simulink subsystem "FlexibleDriveline"  (R2025b)
settings: Solver=VariableStepAuto  StartTime=0.0  StopTime=10.0  RelTol=1e-3
PreLoadFcn:
  | FlexibleDrivelineParams;
undefined symbols (not defined in the file or in its folder): flexDLParams, fs
libraries: fl_lib x41, sdl_lib x24, nesl_utility x3
(part 2 of 2)

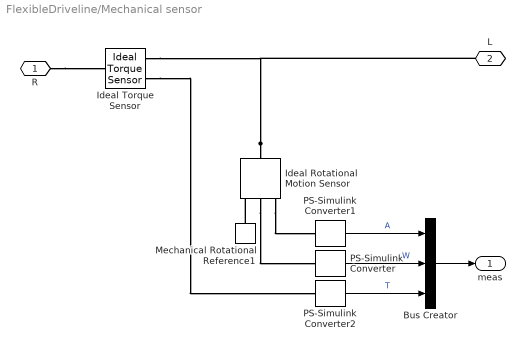
== system FlexibleDriveline/Mechanical sensor ==
  Bus Creator : BusCreator  Inputs=3
  Ideal Rotational Motion Sensor : fl_lib/Mechanical/Mechanical Sensors/Ideal Rotational Motion Sensor  reference=foundation.enum.MeasurementReference.difference  acceleration_port=false  velocity_port=true  position_port=true  wrap_angle=simscape.enum.onoff.off  offset=0 deg
  Ideal Torque Sensor : fl_lib/Mechanical/Mechanical Sensors/Ideal Torque Sensor
  Mechanical Rotational Reference1 : fl_lib/Mechanical/Rotational Elements/Mechanical Rotational Reference
  PS-Simulink Converter : nesl_utility/PS-Simulink Converter  PhysicalDomain=network_engine_domain  SubClassName=ps_output  LeftPortType=input  RightPortType=output  PseudoPeriodic=off  Frequencies=[]  VectorFormat=1-D array  Unit=rad/s  AffineConversion=off
  PS-Simulink Converter1 : nesl_utility/PS-Simulink Converter  PhysicalDomain=network_engine_domain  SubClassName=ps_output  LeftPortType=input  RightPortType=output  PseudoPeriodic=off  Frequencies=[]  VectorFormat=1-D array  Unit=rad  AffineConversion=off
  PS-Simulink Converter2 : nesl_utility/PS-Simulink Converter  PhysicalDomain=network_engine_domain  SubClassName=ps_output  LeftPortType=input  RightPortType=output  PseudoPeriodic=off  Frequencies=[]  VectorFormat=1-D array  Unit=N*m  AffineConversion=off
  R : PMIOPort  Side=Left
  L : PMIOPort  Port=2  Side=Right
  meas : Outport  VectorParamsAs1DForOutWhenUnconnected=off
  wires:
  PS-Simulink Converter2/1 -> Bus Creator/3  "T"
  PS-Simulink Converter/1 -> Bus Creator/2  "W"
  PS-Simulink Converter1/1 -> Bus Creator/1  "A"
  Bus Creator/1 -> meas/1
  connections:
  Mechanical Rotational Reference1/LConn1 -- Ideal Rotational Motion Sensor/RConn1
  Ideal Rotational Motion Sensor/RConn3 -- PS-Simulink Converter1/LConn1
  Ideal Rotational Motion Sensor/RConn2 -- PS-Simulink Converter/LConn1
  Ideal Rotational Motion Sensor/LConn1 -- Ideal Torque Sensor/RConn1 -- L/RConn1
  R/RConn1 -- Ideal Torque Sensor/LConn1
  Ideal Torque Sensor/RConn2 -- PS-Simulink Converter2/LConn1

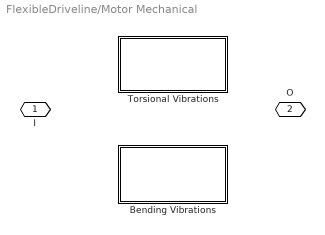
== system FlexibleDriveline/Motor Mechanical ==
  Bending Vibrations : Subsystem  VariantControl=false
  Torsional Vibrations : Subsystem  VariantControl=true
  I : PMIOPort  Side=Left
  O : PMIOPort  Port=2  Side=Right

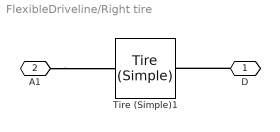
== system FlexibleDriveline/Right tire ==
  Tire (Simple)1 : sdl_lib/Tires & Vehicles/Tire (Simple)  r_tire=flexDLParams.gearBox.tireR m  model_compliance=sdl.enum.compliance.on  stiffness=1e6 N/m  damping=1000 N*s/m  model_inertia=sdl.enum.model_inertia.on  tire_inertia=1 kg*m^2  initial_velocity=0 rad/s
      settings: InternalSimscapePortConfiguration="{\"Bottom\":[],\"Left\":[{\"id\":\"A\",\"label\":\"A\",\"type\":\"foundation.mechanical.rotational.rotational\"}],\"Right\":[{\"id\":\"H\",\"label\":\"H\",\"type\":\"foundation.mechanical.translational.translational\"}],\"Top\":[]}"
  D : PMIOPort  Side=Left
  A1 : PMIOPort  Port=2  Side=Right
  connections:
  A1/RConn1 -- Tire (Simple)1/LConn1
  D/RConn1 -- Tire (Simple)1/RConn1

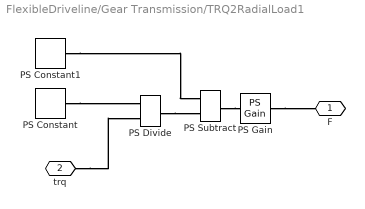
== system FlexibleDriveline/Gear Transmission/TRQ2RadialLoad1 ==
  PS Constant : fl_lib/Physical Signals/Sources/PS Constant  constant=25e-3 m
  PS Constant1 : fl_lib/Physical Signals/Sources/PS Constant  constant=5*9.81 N
  PS Divide : fl_lib/Physical Signals/Functions/PS Divide
  PS Gain : fl_lib/Physical Signals/Functions/PS Gain  gain=0.5
  PS Subtract : fl_lib/Physical Signals/Functions/PS Subtract
  F : PMIOPort  Side=Right
  trq : PMIOPort  Port=2  Side=Left
  connections:
  trq/RConn1 -- PS Divide/LConn1
  PS Constant1/RConn1 -- PS Subtract/LConn2
  PS Divide/RConn1 -- PS Subtract/LConn1
  PS Gain/RConn1 -- F/RConn1
  PS Subtract/RConn1 -- PS Gain/LConn1
  PS Constant/RConn1 -- PS Divide/LConn2

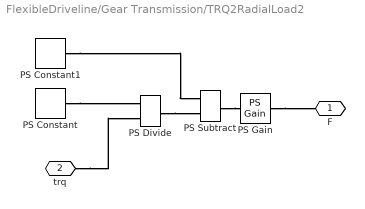
== system FlexibleDriveline/Gear Transmission/TRQ2RadialLoad2 ==
  PS Constant : fl_lib/Physical Signals/Sources/PS Constant  constant=25e-3 m
  PS Constant1 : fl_lib/Physical Signals/Sources/PS Constant  constant=5*9.81 N
  PS Divide : fl_lib/Physical Signals/Functions/PS Divide
  PS Gain : fl_lib/Physical Signals/Functions/PS Gain  gain=0.5
  PS Subtract : fl_lib/Physical Signals/Functions/PS Subtract
  F : PMIOPort  Side=Right
  trq : PMIOPort  Port=2  Side=Left
  connections:
  trq/RConn1 -- PS Divide/LConn1
  PS Constant1/RConn1 -- PS Subtract/LConn2
  PS Divide/RConn1 -- PS Subtract/LConn1
  PS Gain/RConn1 -- F/RConn1
  PS Subtract/RConn1 -- PS Gain/LConn1
  PS Constant/RConn1 -- PS Divide/LConn2

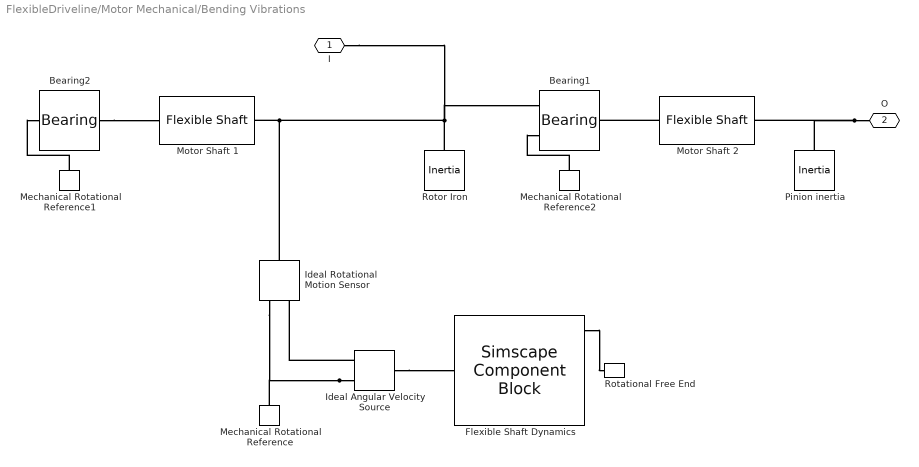
== system FlexibleDriveline/Motor Mechanical/Bending Vibrations ==
  Bearing1 : sdl_lib/Couplings & Drives/Bearing  bearingType=sdl.enum.bearingType.BallRoller  enableFollower=true  casing=true  radius=flexDLParams.motorMech.bearing1ID/2 mm  length=flexDLParams.motorMech.bearing1Length mm  loadType=foundation.enum.constant_variable.constant  load=10 N  F_thr=0.001 N  w_thr=0.001 rev/s  frictionType=foundation.enum.constant_variable.variable  interp_method_1=simscape.enum.interpolation.linear  extrap_method_1=simscape.enum.extrapolation.linear  f_coeff=0.002  N_TLU=flexDLParams.motorMech.speedRPM rpm  f_coeff_TLU=flexDLParams.motorMech.frictionCoff  customizeFrictionCurve=false  mu=0.29 Pa*s  visc_coeff_min=0.002  bearingModulus=7.2519e-08 rev  muN_P_norm_TLU=[.4306, .6124, .6651, .7512, .866, 1, 1.1962, 1.4354, 3.8517]  visc_coeff_norm_TLU=[3.6621, 1.672, 1.3397, 1.1811, 1.0743, 1, 1.0358, 1.1173, 2.2792]  interp_method_2=simscape.enum.interpolation.linear  extrap_method_2=simscape.enum.extrapolation.linear
      settings: InternalSimscapePortConfiguration="{\"Bottom\":[{\"id\":\"C\",\"label\":\"C\",\"type\":\"foundation.mechanical.rotational.rotational\"}],\"Left\":[{\"id\":\"B\",\"label\":\"B\",\"type\":\"foundation.mechanical.rotational.rotational\"}],\"Right\":[{\"id\":\"F\",\"label\":\"F\",\"type\":\"foundation.mechanical.rotational.rotational\"}],\"Top\":[]}"
  Bearing2 : sdl_lib/Couplings & Drives/Bearing  bearingType=sdl.enum.bearingType.BallRoller  enableFollower=false  casing=true  radius=flexDLParams.motorMech.bearing2ID/2 mm  length=flexDLParams.motorMech.bearing1Length mm  loadType=foundation.enum.constant_variable.constant  load=10 N  F_thr=0.001 N  w_thr=0.001 rev/s  frictionType=foundation.enum.constant_variable.variable  interp_method_1=simscape.enum.interpolation.linear  extrap_method_1=simscape.enum.extrapolation.linear  f_coeff=0.002  N_TLU=flexDLParams.motorMech.speedRPM rpm  f_coeff_TLU=flexDLParams.motorMech.frictionCoff  customizeFrictionCurve=false  mu=0.29 Pa*s  visc_coeff_min=0.002  bearingModulus=7.2519e-08 rev  muN_P_norm_TLU=[.4306, .6124, .6651, .7512, .866, 1, 1.1962, 1.4354, 3.8517]  visc_coeff_norm_TLU=[3.6621, 1.672, 1.3397, 1.1811, 1.0743, 1, 1.0358, 1.1173, 2.2792]  interp_method_2=simscape.enum.interpolation.linear  extrap_method_2=simscape.enum.extrapolation.linear
      settings: InternalSimscapePortConfiguration="{\"Bottom\":[{\"id\":\"C\",\"label\":\"C\",\"type\":\"foundation.mechanical.rotational.rotational\"}],\"Left\":[{\"id\":\"B\",\"label\":\"B\",\"type\":\"foundation.mechanical.rotational.rotational\"}],\"Right\":[],\"Top\":[]}"
  Flexible Shaft Dynamics : SimscapeComponentBlock  SourceFile=sdl.couplings.flexible_shaft  ComponentPath=sdl.couplings.flexible_shaft  ComponentVariants="[\"sdl.couplings.flexible_shaft\"]"  ComponentVariantNames="[\"flexible_shaft\"]"  ClassName=flexible_shaft  SchemaVersion=1  modelTorsion=false  modelTransverse=true  n_segments=1  parameterization=sdl.enum.shaftParameterization.MaterialPropertiesVaried  length=fs.length_shaft m  lengths=fs.zShaft m  shaft_stiffness=2e5 N*m/rad  shaft_inertia=0.02 kg*m^2  shaft_stiffnesses=[400000, 200000, 100000] N*m/rad  shaft_inertias=[.025, .02, .015] kg*m^2  eiIN=5e5 Pa*m^4  rhoaIN=19 kg/m  eiINs=[600000, 500000, 400000] Pa*m^4  rhoaINs=[20, 19, 18] kg/m  density=fs.materialDensity kg/m^3  shear_modulus=fs.shear_modulus Pa  elastic_modulus=fs.elasticModulus Pa  shaft_construction=sdl.enum.shaftConstruction.solid  diameter_outer=fs.diameters_outer(1) m  diameter_inner=fs.diameters_inner(1) m  diameter_outers=fs.diametersOuterTLU m  diameter_inners=interp1(fs.z_TLU, fs.diameters_inner_TLU, fs.z_shaft(2:end)) m  damping_ratio=0.01  mu_visc_BF=[0, 0] N*m/(rad/s)  mu_visc=fs.muViscTors N*m/(rad/s)  initial_deflection=0 rad  initial_velocity=0 rpm  num_supports=sdl.enum.num_supports.two  z_support=fs.zSupport m  boundaryB1=sdl.enum.shaftSupport.bearingMatrix_speed  DrotB1_row=fs.bearing.dRot N*m/(rad/s)  DtransB1_row=[20000, -44000, -44000, 350000] N/(m/s)  DtransB1_w_mat=fs.bearing.D N/(m/s)  KrotB1_row=fs.bearing.kRot N*m/rad  KtransB1_row=[1000000, -200000, -300000, 5000000] N/m  KtransB1_w_mat=fs.bearing.K N/m  boundaryI1=sdl.enum.shaftSupport.bearingMatrix_speed  DrotI1_row=fs.bearing.d_rot N*m/(rad/s)  DtransI1_row=[20000, -44000, -44000, 350000] N/(m/s)  DtransI1_w_mat=fs.bearing.D N/(m/s)  KrotI1_row=fs.bearing.k_rot N*m/rad  KtransI1_row=[1000000, -200000, -300000, 5000000] N/m  KtransI1_w_mat=fs.bearing.K N/m  boundaryI2=sdl.enum.shaftSupport.bearingMatrix_speed  DrotI2_row=fs.bearing.d_rot N*m/(rad/s)  DtransI2_row=[20000, -44000, -44000, 350000] N/(m/s)  DtransI2_w_mat=fs.bearing.D N/(m/s)  KrotI2_row=fs.bearing.k_rot N*m/rad  KtransI2_row=[1000000, -200000, -300000, 5000000] N/m  KtransI2_w_mat=fs.bearing.K N/m  boundaryF1=sdl.enum.shaftSupport.free  DrotF1_row=fs.bearing.dRot N*m/(rad/s)  DtransF1_row=[20000, -44000, -44000, 350000] N/(m/s)  DtransF1_w_mat=fs.bearing.D N/(m/s)  KrotF1_row=fs.bearing.kRot N*m/rad  KtransF1_row=[1000000, -200000, -300000, 5000000] N/m  KtransF1_w_mat=fs.bearing.K N/m  bearing_speed=fs.bearingSpeed*fs.excitationPoles rpm  alpha=fs.aDamp 1/s  beta=fs.bDamp s  noDisk=sdl.enum.shaftDisks.disk  zDisk=fs.zMass m  mDiskIN=fs.pointMass kg  IdDiskIN=fs.Id kg*m^2  IpDiskIN=fs.Ip./fs.excitationPoles kg*m^2  enable_static_unbalance=true  offsetMR=fs.excitationLoad./(fs.excitationPoles*fs.wNominalForcing)^2 kg*m  offsetMR_initialAngleIN=0 rad  offsetMassLocation=fs.bearingSpan12/2 m  enable_external_force=false  externalForce=[1, 2] N  externalForceHarmonic=[.5, 2]  externalLoadAngle=[pi / 2, 3 * pi / 4] rad  zExternalLoad=[.25, .75] m  AnalysisMethod=sdl.enum.bendingAnalysisMethod.Eigenmodes  ModeInputMethod=sdl.enum.modeInputMethod.SimscapeDetermined  numModesIn=fs.numModes  mode_speed_dependency=sdl.enum.mode_speed_dependency.Dynamic  OmegaNom=fs.w_shaft_nominal rad/s  wMax=fs.wMax rad/s  dz=fs.dz m  userMode_w=[280, 644, 615, 1285] rad/s  userMode_w_mat=[257, 780, 580, 1560; 280, 644, 615, 1285; 294, 513, 636, 1020] rad/s  userMode_z=[0, .1, .2, .3, .4, .5, .6, .7, .8, .9, 1] m  userMode_shapeX=[.1648, .0086, -.2759, .0162; .1671, .0093, -.2231, .0133; .1691, .01, -.1689, .0102; .1707, .0105, -.1135, .007; .1717, .0108, -.057, .0035; .1721, .0109, 0, 0; .1717, .0108, .057, -.0035; .1707, .0105, .1135, -.007; .1691, .01, .1689, -.0102; .1671, .0093, .2231, -.0133; .1648, .0086, .2759, -.0162]  userMode_shapeX_mat=cat(3, [.1842, .0134, -.3072, .0272; .1863, .0152, -.2482, .0226; .1882, .0169, -.1878, .0176; .1897, .0182, -.1261, .0121; .1906, .019, -.0634, .0062; .191, .0193, 0, 0; .1906, .019, .0634, -.0062; .1897, .0182, .1261, -.0121; .1882, .0169, .1878, -.0176; .1863, .0152, .2482, -.0226; .1842, .0134, .3072, -.0272], [.1648, .0086, -.2759, .0162; .1671, .0093, -.2231, .0133; .1691, .01, -.1689, .0102; .1707, .0105, -.1135, .007; .1717, .0108, -.057, .0035; .1721, .0109, 0, 0; .1717, .0108, .057, -.0035; .1707, .0105, .1135, -.007; .1691, .01, .1689, -.0102; .1671, .0093, .2231, -.0133; .1648, .0086, .2759, -.0162], [.1291, .0046, -.2166, .0082; .131, .0048, -.1751, .0067; .1327, .005, -.1327, .0051; .1341, .0052, -.0891, .0035; .135, .0053, -.0448, .0017; .1353, .0053, 0, 0; .135, .0053, .0448, -.0017; .1341, .0052, .0891, -.0035; .1327, .005, .1327, -.0051; .131, .0048, .1751, -.0067; .1291, .0046, .2166, -.0082])  userMode_shapeY=[.1193, -.1784, -.1997, -.3348; .1209, -.1933, -.1615, -.2751; .1224, -.2068, -.1223, -.2119; .1235, -.2176, -.0821, -.1445; .1243, -.2245, -.0413, -.0734; .1246, -.2269, 0, 0; .1243, -.2245, .0413, .0734; .1235, -.2176, .0821, .1445; .1224, -.2068, .1223, .2119; .1209, -.1933, .1615, .2751; .1193, -.1784, .1997, .3348]  userMode_shapeY_mat=cat(3, [.0885, -.1625, -.1475, -.3301; .0895, -.1847, -.1192, -.2745; .0904, -.2048, -.0902, -.2141; .0911, -.2209, -.0606, -.1475; .0916, -.2313, -.0304, -.0754; .0917, -.2349, 0, 0; .0916, -.2313, .0304, .0754; .0911, -.2209, .0606, .1475; .0904, -.2048, .0902, .2141; .0895, -.1847, .1192, .2745; .0885, -.1625, .1475, .3301], [.1193, -.1784, -.1997, -.3348; .1209, -.1933, -.1615, -.2751; .1224, -.2068, -.1223, -.2119; .1235, -.2176, -.0821, -.1445; .1243, -.2245, -.0413, -.0734; .1246, -.2269, 0, 0; .1243, -.2245, .0413, .0734; .1235, -.2176, .0821, .1445; .1224, -.2068, .1223, .2119; .1209, -.1933, .1615, .2751; .1193, -.1784, .1997, .3348], [.1566, -.1901, -.2628, -.3377; .1589, -.1994, -.2125, -.2753; .161, -.2079, -.1609, -.2103; .1627, -.2146, -.1081, -.1424; .1638, -.219, -.0544, -.0719; .1642, -.2205, 0, 0; .1638, -.219, .0544, .0719; .1627, -.2146, .1081, .1424; .161, -.2079, .1609, .2103; .1589, -.1994, .2125, .2753; .1566, -.1901, .2628, .3377])  eta_lumped_nominal=5e-7  etaDer_lumped_nominal=1e-4  eta_modal_nominal=1  etaDer_modal_nominal=1
      settings: CopyFcn=simscape.sscblock.internal.componentBlockCallback(gcbh,'COPY')  PreCopyFcn=simscape.sscblock.internal.componentBlockCallback(gcbh,'PRECOPY')  PreDeleteFcn=simscape.sscblock.internal.componentBlockCallback(gcbh,'PREDELETE')  InternalSimscapePortConfiguration="{\"Bottom\":[{\"id\":\"Fsupports\",\"label\":\"Fr\",\"type\":\"output\"},{\"id\":\"Msupports\",\"label\":\"M\",\"type\":\"output\"},{\"id\":\"Vsupports\",\"label\":\"V\",\"type\":\"output\"},{\"id\":\"Wsupports\",\"label\":\"W\",\"type\":\"output\"}],\"Left\":[{\"id\":\"B\",\"label\":\"B\",\"type\":\"foundation.mechanical.rotational.rotational\"}],\"Right\":[{\"id\":\"F\",\"label\":\"F\",\"type\":\"foundation.mechanical.rotational.rotational\"}],\"Top\":[]}"
      mask Type: Flexible Shaft
  Ideal Angular Velocity Source : fl_lib/Mechanical/Mechanical Sources/Ideal Angular Velocity Source
  Ideal Rotational Motion Sensor : fl_lib/Mechanical/Mechanical Sensors/Ideal Rotational Motion Sensor  reference=foundation.enum.MeasurementReference.difference  acceleration_port=false  velocity_port=true  position_port=false  wrap_angle=false  offset=0 rad
      settings: InternalSimscapePortConfiguration="{\"Bottom\":[],\"Left\":[{\"id\":\"R\",\"label\":\"R\",\"type\":\"foundation.mechanical.rotational.rotational\"}],\"Right\":[{\"id\":\"C\",\"label\":\"C\",\"type\":\"foundation.mechanical.rotational.rotational\"},{\"id\":\"W\",\"label\":\"W\",\"type\":\"output\"}],\"Top\":[]}"
  Mechanical Rotational Reference : fl_lib/Mechanical/Rotational Elements/Mechanical Rotational Reference
  Mechanical Rotational Reference1 : fl_lib/Mechanical/Rotational Elements/Mechanical Rotational Reference
  Mechanical Rotational Reference2 : fl_lib/Mechanical/Rotational Elements/Mechanical Rotational Reference
  Motor Shaft 1 : sdl_lib/Couplings & Drives/Flexible Shaft  modelTorsion=true  modelTransverse=false  n_segments=1  parameterization=sdl.enum.shaftParameterization.MaterialPropertiesVaried  length=1 m  lengths=[flexDLParams.motorMech.shaftLengthBearing, flexDLParams.motorMech.stackLength, flexDLParams.motorMech.shaftLengthBearing] mm  shaft_stiffness=2e5 N*m/rad  shaft_inertia=0.02 kg*m^2  shaft_stiffnesses=[400000, 200000, 100000] N*m/rad  shaft_inertias=[.025, .02, .015] kg*m^2  eiIN=5e5 Pa*m^4  rhoaIN=19 kg/m  eiINs=[600000, 500000, 400000] Pa*m^4  rhoaINs=[20, 19, 18] kg/m  density=7.8e3 kg/m^3  shear_modulus=7.93e9 Pa  elastic_modulus=200e9 Pa  shaft_construction=sdl.enum.shaftConstruction.solid  diameter_outer=0.075 m  diameter_inner=0.05 m  diameter_outers=[flexDLParams.motorMech.bearing1ID, flexDLParams.motorMech.shaftDiaAtRotor, flexDLParams.motorMech.bearing2ID] mm  diameter_inners=[.055, .05, .045] m  damping_ratio=0.01  mu_visc_BF=[0, 0] N*m*s/rad  mu_visc=[0, 0] N*m*s/rad  initial_deflection=0 rad  initial_velocity=0 rpm  num_supports=sdl.enum.num_supports.two  z_support=[0, flexDLParams.motorMech.bearingSpan12] mm  boundaryB1=sdl.enum.shaftSupport.clamp  DrotB1_row=[1000, 1000] N*m*s/rad  DtransB1_row=[20000, -44000, -44000, 350000] N*s/m  DtransB1_w_mat=[20000, -44000, -44000, 350000; 10000, -25000, -25000, 140000; 5000, -10000, -10000, 20000] N*s/m  KrotB1_row=[10000, 10000] N*m/rad  KtransB1_row=[1000000, -200000, -300000, 5000000] N/m  KtransB1_w_mat=[1000000, -600000, -3500000, 8000000; 1000000, -200000, -3000000, 5000000; 1000000, -50000, -2500000, 3000000] N/m  boundaryI1=sdl.enum.shaftSupport.clamp  DrotI1_row=[1000, 1000] N*m*s/rad  DtransI1_row=[20000, -44000, -44000, 350000] N*s/m  DtransI1_w_mat=[20000, -44000, -44000, 350000; 10000, -25000, -25000, 140000; 5000, -10000, -10000, 20000] N*s/m  KrotI1_row=[10000, 10000] N*m/rad  KtransI1_row=[1000000, -200000, -300000, 5000000] N/m  KtransI1_w_mat=[1000000, -600000, -3500000, 8000000; 1000000, -200000, -3000000, 5000000; 1000000, -50000, -2500000, 3000000] N/m  boundaryI2=sdl.enum.shaftSupport.clamp  DrotI2_row=[1000, 1000] N*m*s/rad  DtransI2_row=[20000, -44000, -44000, 350000] N*s/m  DtransI2_w_mat=[20000, -44000, -44000, 350000; 10000, -25000, -25000, 140000; 5000, -10000, -10000, 20000] N*s/m  KrotI2_row=[10000, 10000] N*m/rad  KtransI2_row=[1000000, -200000, -300000, 5000000] N/m  KtransI2_w_mat=[1000000, -600000, -3500000, 8000000; 1000000, -200000, -3000000, 5000000; 1000000, -50000, -2500000, 3000000] N/m  boundaryF1=sdl.enum.shaftSupport.clamp  DrotF1_row=[1000, 1000] N*m*s/rad  DtransF1_row=[20000, -44000, -44000, 350000] N*s/m  DtransF1_w_mat=[20000, -44000, -44000, 350000; 10000, -25000, -25000, 140000; 5000, -10000, -10000, 20000] N*s/m  KrotF1_row=[10000, 10000] N*m/rad  KtransF1_row=[1000000, -200000, -300000, 5000000] N/m  KtransF1_w_mat=[1000000, -600000, -3500000, 8000000; 1000000, -200000, -3000000, 5000000; 1000000, -50000, -2500000, 3000000] N/m  bearing_speed=[200, 500, 1500] rpm  alpha=10 1/s  beta=1e-8 s  noDisk=sdl.enum.shaftDisks.none  zDisk=0.5 m  mDiskIN=2 kg  IdDiskIN=0.025 kg*m^2  IpDiskIN=0.050 kg*m^2  enable_static_unbalance=true  offsetMR=[.01, .01] kg*m  offsetMR_initialAngleIN=[0, pi] rad  offsetMassLocation=[.33, .67] m  enable_external_force=false  externalForce=[1, 2] N  externalForceHarmonic=[.5, 2]  externalLoadAngle=[pi / 2, 3 * pi / 4] rad  zExternalLoad=[.25, .75] m  AnalysisMethod=sdl.enum.bendingAnalysisMethod.LumpedMass  ModeInputMethod=sdl.enum.modeInputMethod.SimscapeDetermined  numModesIn=6  mode_speed_dependency=sdl.enum.mode_speed_dependency.Static  OmegaNom=5000 rpm  wMax=1e8 rpm  dz=0.01 m  userMode_w=[280, 644, 615, 1285] rad/s  userMode_w_mat=[257, 780, 580, 1560; 280, 644, 615, 1285; 294, 513, 636, 1020] rad/s  userMode_z=[0, .1, .2, .3, .4, .5, .6, .7, .8, .9, 1] m  userMode_shapeX=[.1648, .0086, -.2759, .0162; .1671, .0093, -.2231, .0133; .1691, .01, -.1689, .0102; .1707, .0105, -.1135, .007; .1717, .0108, -.057, .0035; .1721, .0109, 0, 0; .1717, .0108, .057, -.0035; .1707, .0105, .1135, -.007; .1691, .01, .1689, -.0102; .1671, .0093, .2231, -.0133; .1648, .0086, .2759, -.0162]  userMode_shapeX_mat=cat(3, [.1842, .0134, -.3072, .0272; .1863, .0152, -.2482, .0226; .1882, .0169, -.1878, .0176; .1897, .0182, -.1261, .0121; .1906, .019, -.0634, .0062; .191, .0193, 0, 0; .1906, .019, .0634, -.0062; .1897, .0182, .1261, -.0121; .1882, .0169, .1878, -.0176; .1863, .0152, .2482, -.0226; .1842, .0134, .3072, -.0272], [.1648, .0086, -.2759, .0162; .1671, .0093, -.2231, .0133; .1691, .01, -.1689, .0102; .1707, .0105, -.1135, .007; .1717, .0108, -.057, .0035; .1721, .0109, 0, 0; .1717, .0108, .057, -.0035; .1707, .0105, .1135, -.007; .1691, .01, .1689, -.0102; .1671, .0093, .2231, -.0133; .1648, .0086, .2759, -.0162], [.1291, .0046, -.2166, .0082; .131, .0048, -.1751, .0067; .1327, .005, -.1327, .0051; .1341, .0052, -.0891, .0035; .135, .0053, -.0448, .0017; .1353, .0053, 0, 0; .135, .0053, .0448, -.0017; .1341, .0052, .0891, -.0035; .1327, .005, .1327, -.0051; .131, .0048, .1751, -.0067; .1291, .0046, .2166, -.0082])  userMode_shapeY=[.1193, -.1784, -.1997, -.3348; .1209, -.1933, -.1615, -.2751; .1224, -.2068, -.1223, -.2119; .1235, -.2176, -.0821, -.1445; .1243, -.2245, -.0413, -.0734; .1246, -.2269, 0, 0; .1243, -.2245, .0413, .0734; .1235, -.2176, .0821, .1445; .1224, -.2068, .1223, .2119; .1209, -.1933, .1615, .2751; .1193, -.1784, .1997, .3348]  userMode_shapeY_mat=cat(3, [.0885, -.1625, -.1475, -.3301; .0895, -.1847, -.1192, -.2745; .0904, -.2048, -.0902, -.2141; .0911, -.2209, -.0606, -.1475; .0916, -.2313, -.0304, -.0754; .0917, -.2349, 0, 0; .0916, -.2313, .0304, .0754; .0911, -.2209, .0606, .1475; .0904, -.2048, .0902, .2141; .0895, -.1847, .1192, .2745; .0885, -.1625, .1475, .3301], [.1193, -.1784, -.1997, -.3348; .1209, -.1933, -.1615, -.2751; .1224, -.2068, -.1223, -.2119; .1235, -.2176, -.0821, -.1445; .1243, -.2245, -.0413, -.0734; .1246, -.2269, 0, 0; .1243, -.2245, .0413, .0734; .1235, -.2176, .0821, .1445; .1224, -.2068, .1223, .2119; .1209, -.1933, .1615, .2751; .1193, -.1784, .1997, .3348], [.1566, -.1901, -.2628, -.3377; .1589, -.1994, -.2125, -.2753; .161, -.2079, -.1609, -.2103; .1627, -.2146, -.1081, -.1424; .1638, -.219, -.0544, -.0719; .1642, -.2205, 0, 0; .1638, -.219, .0544, .0719; .1627, -.2146, .1081, .1424; .161, -.2079, .1609, .2103; .1589, -.1994, .2125, .2753; .1566, -.1901, .2628, .3377])  eta_lumped_nominal=1  etaDer_lumped_nominal=1  eta_modal_nominal=1  etaDer_modal_nominal=1
      settings: InternalSimscapePortConfiguration="{\"Bottom\":[],\"Left\":[{\"id\":\"B\",\"label\":\"B\",\"type\":\"foundation.mechanical.rotational.rotational\"}],\"Right\":[{\"id\":\"F\",\"label\":\"F\",\"type\":\"foundation.mechanical.rotational.rotational\"}],\"Top\":[]}"
  Motor Shaft 2 : sdl_lib/Couplings & Drives/Flexible Shaft  modelTorsion=true  modelTransverse=false  n_segments=1  parameterization=sdl.enum.shaftParameterization.MaterialProperties  length=flexDLParams.motorMech.shaftOverHang mm  lengths=[1, .5, .25] m  shaft_stiffness=2e5 N*m/rad  shaft_inertia=0.02 kg*m^2  shaft_stiffnesses=[400000, 200000, 100000] N*m/rad  shaft_inertias=[.025, .02, .015] kg*m^2  eiIN=5e5 Pa*m^4  rhoaIN=19 kg/m  eiINs=[600000, 500000, 400000] Pa*m^4  rhoaINs=[20, 19, 18] kg/m  density=7.8e3 kg/m^3  shear_modulus=7.93e9 Pa  elastic_modulus=200e9 Pa  shaft_construction=sdl.enum.shaftConstruction.solid  diameter_outer=flexDLParams.motorMech.bearing2ID mm  diameter_inner=0.05 m  diameter_outers=[.085, .075, .065] m  diameter_inners=[.055, .05, .045] m  damping_ratio=0.01  mu_visc_BF=[0, 0] N*m*s/rad  mu_visc=[0, 0] N*m*s/rad  initial_deflection=0 rad  initial_velocity=0 rpm  num_supports=sdl.enum.num_supports.two  z_support=[0, flexDLParams.motorMech.bearing1Length] mm  boundaryB1=sdl.enum.shaftSupport.clamp  DrotB1_row=[1000, 1000] N*m*s/rad  DtransB1_row=[20000, -44000, -44000, 350000] N*s/m  DtransB1_w_mat=[20000, -44000, -44000, 350000; 10000, -25000, -25000, 140000; 5000, -10000, -10000, 20000] N*s/m  KrotB1_row=[10000, 10000] N*m/rad  KtransB1_row=[1000000, -200000, -300000, 5000000] N/m  KtransB1_w_mat=[1000000, -600000, -3500000, 8000000; 1000000, -200000, -3000000, 5000000; 1000000, -50000, -2500000, 3000000] N/m  boundaryI1=sdl.enum.shaftSupport.clamp  DrotI1_row=[1000, 1000] N*m*s/rad  DtransI1_row=[20000, -44000, -44000, 350000] N*s/m  DtransI1_w_mat=[20000, -44000, -44000, 350000; 10000, -25000, -25000, 140000; 5000, -10000, -10000, 20000] N*s/m  KrotI1_row=[10000, 10000] N*m/rad  KtransI1_row=[1000000, -200000, -300000, 5000000] N/m  KtransI1_w_mat=[1000000, -600000, -3500000, 8000000; 1000000, -200000, -3000000, 5000000; 1000000, -50000, -2500000, 3000000] N/m  boundaryI2=sdl.enum.shaftSupport.clamp  DrotI2_row=[1000, 1000] N*m*s/rad  DtransI2_row=[20000, -44000, -44000, 350000] N*s/m  DtransI2_w_mat=[20000, -44000, -44000, 350000; 10000, -25000, -25000, 140000; 5000, -10000, -10000, 20000] N*s/m  KrotI2_row=[10000, 10000] N*m/rad  KtransI2_row=[1000000, -200000, -300000, 5000000] N/m  KtransI2_w_mat=[1000000, -600000, -3500000, 8000000; 1000000, -200000, -3000000, 5000000; 1000000, -50000, -2500000, 3000000] N/m  boundaryF1=sdl.enum.shaftSupport.clamp  DrotF1_row=[1000, 1000] N*m*s/rad  DtransF1_row=[20000, -44000, -44000, 350000] N*s/m  DtransF1_w_mat=[20000, -44000, -44000, 350000; 10000, -25000, -25000, 140000; 5000, -10000, -10000, 20000] N*s/m  KrotF1_row=[10000, 10000] N*m/rad  KtransF1_row=[1000000, -200000, -300000, 5000000] N/m  KtransF1_w_mat=[1000000, -600000, -3500000, 8000000; 1000000, -200000, -3000000, 5000000; 1000000, -50000, -2500000, 3000000] N/m  bearing_speed=[200, 500, 1500] rpm  alpha=10 1/s  beta=1e-8 s  noDisk=sdl.enum.shaftDisks.none  zDisk=0.5 m  mDiskIN=2 kg  IdDiskIN=0.025 kg*m^2  IpDiskIN=0.050 kg*m^2  enable_static_unbalance=true  offsetMR=[.01, .01] kg*m  offsetMR_initialAngleIN=[0, pi] rad  offsetMassLocation=[.33, .67] m  enable_external_force=false  externalForce=[1, 2] N  externalForceHarmonic=[.5, 2]  externalLoadAngle=[pi / 2, 3 * pi / 4] rad  zExternalLoad=[.25, .75] m  AnalysisMethod=sdl.enum.bendingAnalysisMethod.LumpedMass  ModeInputMethod=sdl.enum.modeInputMethod.SimscapeDetermined  numModesIn=6  mode_speed_dependency=sdl.enum.mode_speed_dependency.Static  OmegaNom=5000 rpm  wMax=1e8 rpm  dz=0.01 m  userMode_w=[280, 644, 615, 1285] rad/s  userMode_w_mat=[257, 780, 580, 1560; 280, 644, 615, 1285; 294, 513, 636, 1020] rad/s  userMode_z=[0, .1, .2, .3, .4, .5, .6, .7, .8, .9, 1] m  userMode_shapeX=[.1648, .0086, -.2759, .0162; .1671, .0093, -.2231, .0133; .1691, .01, -.1689, .0102; .1707, .0105, -.1135, .007; .1717, .0108, -.057, .0035; .1721, .0109, 0, 0; .1717, .0108, .057, -.0035; .1707, .0105, .1135, -.007; .1691, .01, .1689, -.0102; .1671, .0093, .2231, -.0133; .1648, .0086, .2759, -.0162]  userMode_shapeX_mat=cat(3, [.1842, .0134, -.3072, .0272; .1863, .0152, -.2482, .0226; .1882, .0169, -.1878, .0176; .1897, .0182, -.1261, .0121; .1906, .019, -.0634, .0062; .191, .0193, 0, 0; .1906, .019, .0634, -.0062; .1897, .0182, .1261, -.0121; .1882, .0169, .1878, -.0176; .1863, .0152, .2482, -.0226; .1842, .0134, .3072, -.0272], [.1648, .0086, -.2759, .0162; .1671, .0093, -.2231, .0133; .1691, .01, -.1689, .0102; .1707, .0105, -.1135, .007; .1717, .0108, -.057, .0035; .1721, .0109, 0, 0; .1717, .0108, .057, -.0035; .1707, .0105, .1135, -.007; .1691, .01, .1689, -.0102; .1671, .0093, .2231, -.0133; .1648, .0086, .2759, -.0162], [.1291, .0046, -.2166, .0082; .131, .0048, -.1751, .0067; .1327, .005, -.1327, .0051; .1341, .0052, -.0891, .0035; .135, .0053, -.0448, .0017; .1353, .0053, 0, 0; .135, .0053, .0448, -.0017; .1341, .0052, .0891, -.0035; .1327, .005, .1327, -.0051; .131, .0048, .1751, -.0067; .1291, .0046, .2166, -.0082])  userMode_shapeY=[.1193, -.1784, -.1997, -.3348; .1209, -.1933, -.1615, -.2751; .1224, -.2068, -.1223, -.2119; .1235, -.2176, -.0821, -.1445; .1243, -.2245, -.0413, -.0734; .1246, -.2269, 0, 0; .1243, -.2245, .0413, .0734; .1235, -.2176, .0821, .1445; .1224, -.2068, .1223, .2119; .1209, -.1933, .1615, .2751; .1193, -.1784, .1997, .3348]  userMode_shapeY_mat=cat(3, [.0885, -.1625, -.1475, -.3301; .0895, -.1847, -.1192, -.2745; .0904, -.2048, -.0902, -.2141; .0911, -.2209, -.0606, -.1475; .0916, -.2313, -.0304, -.0754; .0917, -.2349, 0, 0; .0916, -.2313, .0304, .0754; .0911, -.2209, .0606, .1475; .0904, -.2048, .0902, .2141; .0895, -.1847, .1192, .2745; .0885, -.1625, .1475, .3301], [.1193, -.1784, -.1997, -.3348; .1209, -.1933, -.1615, -.2751; .1224, -.2068, -.1223, -.2119; .1235, -.2176, -.0821, -.1445; .1243, -.2245, -.0413, -.0734; .1246, -.2269, 0, 0; .1243, -.2245, .0413, .0734; .1235, -.2176, .0821, .1445; .1224, -.2068, .1223, .2119; .1209, -.1933, .1615, .2751; .1193, -.1784, .1997, .3348], [.1566, -.1901, -.2628, -.3377; .1589, -.1994, -.2125, -.2753; .161, -.2079, -.1609, -.2103; .1627, -.2146, -.1081, -.1424; .1638, -.219, -.0544, -.0719; .1642, -.2205, 0, 0; .1638, -.219, .0544, .0719; .1627, -.2146, .1081, .1424; .161, -.2079, .1609, .2103; .1589, -.1994, .2125, .2753; .1566, -.1901, .2628, .3377])  eta_lumped_nominal=1  etaDer_lumped_nominal=1  eta_modal_nominal=1  etaDer_modal_nominal=1
      settings: InternalSimscapePortConfiguration="{\"Bottom\":[],\"Left\":[{\"id\":\"B\",\"label\":\"B\",\"type\":\"foundation.mechanical.rotational.rotational\"}],\"Right\":[{\"id\":\"F\",\"label\":\"F\",\"type\":\"foundation.mechanical.rotational.rotational\"}],\"Top\":[]}"
  Pinion inertia : fl_lib/Mechanical/Rotational Elements/Inertia  inertia=flexDLParams.motor.j*0.2 kg*m^2  num_ports=foundation.enum.numPorts2.one  w_specify=on  w_priority=High  w=0 rpm  w_nominal_specify=off  w_nominal_value=1  w_nominal_unit=rad/s  t_specify=off  t_priority=High  t=0 N*m  t_nominal_specify=off  t_nominal_value=1  t_nominal_unit=N*m
  Rotational Free End : fl_lib/Mechanical/Rotational Elements/Rotational Free End  w_specify=off  w_priority=None  w=0 rad/s  w_nominal_specify=off  w_nominal_value=1  w_nominal_unit=rad/s
  Rotor Iron : fl_lib/Mechanical/Rotational Elements/Inertia  inertia=flexDLParams.motor.j*0.5 kg*m^2  num_ports=foundation.enum.numPorts2.one  w_specify=on  w_priority=High  w=0 rpm  w_nominal_specify=off  w_nominal_value=1  w_nominal_unit=rad/s  t_specify=off  t_priority=High  t=0 N*m  t_nominal_specify=off  t_nominal_value=1  t_nominal_unit=N*m
  I : PMIOPort  Side=Left
  O : PMIOPort  Port=2  Side=Right
  connections:
  Bearing2/LConn1 -- Motor Shaft 1/LConn1
  Mechanical Rotational Reference1/LConn1 -- Bearing2/RConn1
  Motor Shaft 2/LConn1 -- Bearing1/LConn1
  I/RConn1 -- Bearing1/RConn1 -- Rotor Iron/LConn1 -- Motor Shaft 1/RConn1 -- Ideal Rotational Motion Sensor/LConn1
  Mechanical Rotational Reference2/LConn1 -- Bearing1/RConn2
  O/RConn1 -- Motor Shaft 2/RConn1 -- Pinion inertia/LConn1
  Ideal Angular Velocity Source/RConn1 -- Ideal Rotational Motion Sensor/RConn2
  Ideal Angular Velocity Source/LConn1 -- Flexible Shaft Dynamics/LConn1
  Flexible Shaft Dynamics/RConn1 -- Rotational Free End/LConn1
  Ideal Angular Velocity Source/RConn2 -- Ideal Rotational Motion Sensor/RConn1 -- Mechanical Rotational Reference/LConn1

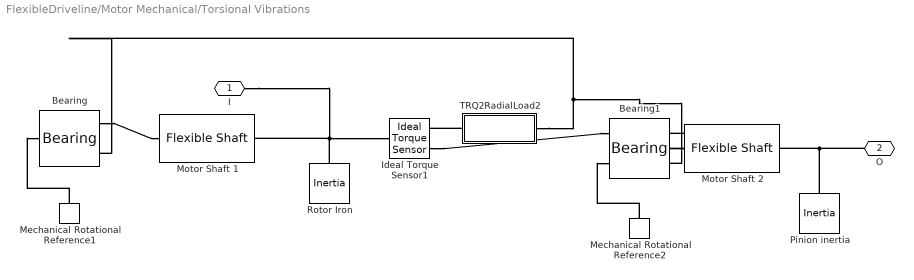
== system FlexibleDriveline/Motor Mechanical/Torsional Vibrations ==
  Bearing : sdl_lib/Couplings & Drives/Bearing  bearingType=sdl.enum.bearingType.BallRoller  enableFollower=false  casing=true  radius=flexDLParams.motorMech.bearing1ID/2 mm  length=flexDLParams.motorMech.bearing1Length mm  loadType=foundation.enum.constant_variable.variable  load=10 N  F_thr=0.001 N  w_thr=0.001 rev/s  frictionType=foundation.enum.constant_variable.variable  interp_method_1=simscape.enum.interpolation.linear  extrap_method_1=simscape.enum.extrapolation.linear  f_coeff=0.002  N_TLU=flexDLParams.motorMech.speedRPM rpm  f_coeff_TLU=flexDLParams.motorMech.frictionCoff  customizeFrictionCurve=false  mu=0.29 Pa*s  visc_coeff_min=0.002  bearingModulus=7.2519e-08 rev  muN_P_norm_TLU=[.4306, .6124, .6651, .7512, .866, 1, 1.1962, 1.4354, 3.8517]  visc_coeff_norm_TLU=[3.6621, 1.672, 1.3397, 1.1811, 1.0743, 1, 1.0358, 1.1173, 2.2792]  interp_method_2=simscape.enum.interpolation.linear  extrap_method_2=simscape.enum.extrapolation.linear
      settings: InternalSimscapePortConfiguration="{\"Bottom\":[{\"id\":\"C\",\"label\":\"C\",\"type\":\"foundation.mechanical.rotational.rotational\"}],\"Left\":[{\"id\":\"B\",\"label\":\"B\",\"type\":\"foundation.mechanical.rotational.rotational\"}],\"Right\":[],\"Top\":[{\"id\":\"Force\",\"label\":\"Load\",\"type\":\"input\"}]}"
  Bearing1 : sdl_lib/Couplings & Drives/Bearing  bearingType=sdl.enum.bearingType.BallRoller  enableFollower=true  casing=true  radius=flexDLParams.motorMech.bearing1ID/2 mm  length=flexDLParams.motorMech.bearing1Length mm  loadType=foundation.enum.constant_variable.variable  load=10 N  F_thr=0.001 N  w_thr=0.001 rev/s  frictionType=foundation.enum.constant_variable.variable  interp_method_1=simscape.enum.interpolation.linear  extrap_method_1=simscape.enum.extrapolation.linear  f_coeff=0.002  N_TLU=flexDLParams.motorMech.speedRPM rpm  f_coeff_TLU=flexDLParams.motorMech.frictionCoff  customizeFrictionCurve=false  mu=0.29 Pa*s  visc_coeff_min=0.002  bearingModulus=7.2519e-08 rev  muN_P_norm_TLU=[.4306, .6124, .6651, .7512, .866, 1, 1.1962, 1.4354, 3.8517]  visc_coeff_norm_TLU=[3.6621, 1.672, 1.3397, 1.1811, 1.0743, 1, 1.0358, 1.1173, 2.2792]  interp_method_2=simscape.enum.interpolation.linear  extrap_method_2=simscape.enum.extrapolation.linear
      settings: InternalSimscapePortConfiguration="{\"Bottom\":[{\"id\":\"C\",\"label\":\"C\",\"type\":\"foundation.mechanical.rotational.rotational\"}],\"Left\":[{\"id\":\"B\",\"label\":\"B\",\"type\":\"foundation.mechanical.rotational.rotational\"}],\"Right\":[{\"id\":\"F\",\"label\":\"F\",\"type\":\"foundation.mechanical.rotational.rotational\"}],\"Top\":[{\"id\":\"Force\",\"label\":\"Load\",\"type\":\"input\"}]}"
  Ideal Torque Sensor1 : fl_lib/Mechanical/Mechanical Sensors/Ideal Torque Sensor
  Mechanical Rotational Reference1 : fl_lib/Mechanical/Rotational Elements/Mechanical Rotational Reference
  Mechanical Rotational Reference2 : fl_lib/Mechanical/Rotational Elements/Mechanical Rotational Reference
  Motor Shaft 1 : sdl_lib/Couplings & Drives/Flexible Shaft  modelTorsion=true  modelTransverse=false  n_segments=1  parameterization=sdl.enum.shaftParameterization.MaterialPropertiesVaried  length=1 m  lengths=[flexDLParams.motorMech.shaftLengthBearing, flexDLParams.motorMech.stackLength, flexDLParams.motorMech.shaftLengthBearing] mm  shaft_stiffness=2e5 N*m/rad  shaft_inertia=0.02 kg*m^2  shaft_stiffnesses=[400000, 200000, 100000] N*m/rad  shaft_inertias=[.025, .02, .015] kg*m^2  eiIN=5e5 Pa*m^4  rhoaIN=19 kg/m  eiINs=[600000, 500000, 400000] Pa*m^4  rhoaINs=[20, 19, 18] kg/m  density=7.8e3 kg/m^3  shear_modulus=7.93e9 Pa  elastic_modulus=200e9 Pa  shaft_construction=sdl.enum.shaftConstruction.solid  diameter_outer=0.075 m  diameter_inner=0.05 m  diameter_outers=[flexDLParams.motorMech.bearing1ID, flexDLParams.motorMech.shaftDiaAtRotor, flexDLParams.motorMech.bearing2ID] mm  diameter_inners=[.055, .05, .045] m  damping_ratio=0.01  mu_visc_BF=[0, 0] N*m*s/rad  mu_visc=[0, 0] N*m*s/rad  initial_deflection=0 rad  initial_velocity=0 rpm  num_supports=sdl.enum.num_supports.two  z_support=[0, flexDLParams.motorMech.bearingSpan12] mm  boundaryB1=sdl.enum.shaftSupport.clamp  DrotB1_row=[1000, 1000] N*m*s/rad  DtransB1_row=[20000, -44000, -44000, 350000] N*s/m  DtransB1_w_mat=[20000, -44000, -44000, 350000; 10000, -25000, -25000, 140000; 5000, -10000, -10000, 20000] N*s/m  KrotB1_row=[10000, 10000] N*m/rad  KtransB1_row=[1000000, -200000, -300000, 5000000] N/m  KtransB1_w_mat=[1000000, -600000, -3500000, 8000000; 1000000, -200000, -3000000, 5000000; 1000000, -50000, -2500000, 3000000] N/m  boundaryI1=sdl.enum.shaftSupport.clamp  DrotI1_row=[1000, 1000] N*m*s/rad  DtransI1_row=[20000, -44000, -44000, 350000] N*s/m  DtransI1_w_mat=[20000, -44000, -44000, 350000; 10000, -25000, -25000, 140000; 5000, -10000, -10000, 20000] N*s/m  KrotI1_row=[10000, 10000] N*m/rad  KtransI1_row=[1000000, -200000, -300000, 5000000] N/m  KtransI1_w_mat=[1000000, -600000, -3500000, 8000000; 1000000, -200000, -3000000, 5000000; 1000000, -50000, -2500000, 3000000] N/m  boundaryI2=sdl.enum.shaftSupport.clamp  DrotI2_row=[1000, 1000] N*m*s/rad  DtransI2_row=[20000, -44000, -44000, 350000] N*s/m  DtransI2_w_mat=[20000, -44000, -44000, 350000; 10000, -25000, -25000, 140000; 5000, -10000, -10000, 20000] N*s/m  KrotI2_row=[10000, 10000] N*m/rad  KtransI2_row=[1000000, -200000, -300000, 5000000] N/m  KtransI2_w_mat=[1000000, -600000, -3500000, 8000000; 1000000, -200000, -3000000, 5000000; 1000000, -50000, -2500000, 3000000] N/m  boundaryF1=sdl.enum.shaftSupport.clamp  DrotF1_row=[1000, 1000] N*m*s/rad  DtransF1_row=[20000, -44000, -44000, 350000] N*s/m  DtransF1_w_mat=[20000, -44000, -44000, 350000; 10000, -25000, -25000, 140000; 5000, -10000, -10000, 20000] N*s/m  KrotF1_row=[10000, 10000] N*m/rad  KtransF1_row=[1000000, -200000, -300000, 5000000] N/m  KtransF1_w_mat=[1000000, -600000, -3500000, 8000000; 1000000, -200000, -3000000, 5000000; 1000000, -50000, -2500000, 3000000] N/m  bearing_speed=[200, 500, 1500] rpm  alpha=10 1/s  beta=1e-8 s  noDisk=sdl.enum.shaftDisks.none  zDisk=0.5 m  mDiskIN=2 kg  IdDiskIN=0.025 kg*m^2  IpDiskIN=0.050 kg*m^2  enable_static_unbalance=true  offsetMR=[.01, .01] kg*m  offsetMR_initialAngleIN=[0, pi] rad  offsetMassLocation=[.33, .67] m  enable_external_force=false  externalForce=[1, 2] N  externalForceHarmonic=[.5, 2]  externalLoadAngle=[pi / 2, 3 * pi / 4] rad  zExternalLoad=[.25, .75] m  AnalysisMethod=sdl.enum.bendingAnalysisMethod.LumpedMass  ModeInputMethod=sdl.enum.modeInputMethod.SimscapeDetermined  numModesIn=6  mode_speed_dependency=sdl.enum.mode_speed_dependency.Static  OmegaNom=5000 rpm  wMax=1e8 rpm  dz=0.01 m  userMode_w=[280, 644, 615, 1285] rad/s  userMode_w_mat=[257, 780, 580, 1560; 280, 644, 615, 1285; 294, 513, 636, 1020] rad/s  userMode_z=[0, .1, .2, .3, .4, .5, .6, .7, .8, .9, 1] m  userMode_shapeX=[.1648, .0086, -.2759, .0162; .1671, .0093, -.2231, .0133; .1691, .01, -.1689, .0102; .1707, .0105, -.1135, .007; .1717, .0108, -.057, .0035; .1721, .0109, 0, 0; .1717, .0108, .057, -.0035; .1707, .0105, .1135, -.007; .1691, .01, .1689, -.0102; .1671, .0093, .2231, -.0133; .1648, .0086, .2759, -.0162]  userMode_shapeX_mat=cat(3, [.1842, .0134, -.3072, .0272; .1863, .0152, -.2482, .0226; .1882, .0169, -.1878, .0176; .1897, .0182, -.1261, .0121; .1906, .019, -.0634, .0062; .191, .0193, 0, 0; .1906, .019, .0634, -.0062; .1897, .0182, .1261, -.0121; .1882, .0169, .1878, -.0176; .1863, .0152, .2482, -.0226; .1842, .0134, .3072, -.0272], [.1648, .0086, -.2759, .0162; .1671, .0093, -.2231, .0133; .1691, .01, -.1689, .0102; .1707, .0105, -.1135, .007; .1717, .0108, -.057, .0035; .1721, .0109, 0, 0; .1717, .0108, .057, -.0035; .1707, .0105, .1135, -.007; .1691, .01, .1689, -.0102; .1671, .0093, .2231, -.0133; .1648, .0086, .2759, -.0162], [.1291, .0046, -.2166, .0082; .131, .0048, -.1751, .0067; .1327, .005, -.1327, .0051; .1341, .0052, -.0891, .0035; .135, .0053, -.0448, .0017; .1353, .0053, 0, 0; .135, .0053, .0448, -.0017; .1341, .0052, .0891, -.0035; .1327, .005, .1327, -.0051; .131, .0048, .1751, -.0067; .1291, .0046, .2166, -.0082])  userMode_shapeY=[.1193, -.1784, -.1997, -.3348; .1209, -.1933, -.1615, -.2751; .1224, -.2068, -.1223, -.2119; .1235, -.2176, -.0821, -.1445; .1243, -.2245, -.0413, -.0734; .1246, -.2269, 0, 0; .1243, -.2245, .0413, .0734; .1235, -.2176, .0821, .1445; .1224, -.2068, .1223, .2119; .1209, -.1933, .1615, .2751; .1193, -.1784, .1997, .3348]  userMode_shapeY_mat=cat(3, [.0885, -.1625, -.1475, -.3301; .0895, -.1847, -.1192, -.2745; .0904, -.2048, -.0902, -.2141; .0911, -.2209, -.0606, -.1475; .0916, -.2313, -.0304, -.0754; .0917, -.2349, 0, 0; .0916, -.2313, .0304, .0754; .0911, -.2209, .0606, .1475; .0904, -.2048, .0902, .2141; .0895, -.1847, .1192, .2745; .0885, -.1625, .1475, .3301], [.1193, -.1784, -.1997, -.3348; .1209, -.1933, -.1615, -.2751; .1224, -.2068, -.1223, -.2119; .1235, -.2176, -.0821, -.1445; .1243, -.2245, -.0413, -.0734; .1246, -.2269, 0, 0; .1243, -.2245, .0413, .0734; .1235, -.2176, .0821, .1445; .1224, -.2068, .1223, .2119; .1209, -.1933, .1615, .2751; .1193, -.1784, .1997, .3348], [.1566, -.1901, -.2628, -.3377; .1589, -.1994, -.2125, -.2753; .161, -.2079, -.1609, -.2103; .1627, -.2146, -.1081, -.1424; .1638, -.219, -.0544, -.0719; .1642, -.2205, 0, 0; .1638, -.219, .0544, .0719; .1627, -.2146, .1081, .1424; .161, -.2079, .1609, .2103; .1589, -.1994, .2125, .2753; .1566, -.1901, .2628, .3377])  eta_lumped_nominal=1  etaDer_lumped_nominal=1  eta_modal_nominal=1  etaDer_modal_nominal=1
      settings: InternalSimscapePortConfiguration="{\"Bottom\":[],\"Left\":[{\"id\":\"B\",\"label\":\"B\",\"type\":\"foundation.mechanical.rotational.rotational\"}],\"Right\":[{\"id\":\"F\",\"label\":\"F\",\"type\":\"foundation.mechanical.rotational.rotational\"}],\"Top\":[]}"
  Motor Shaft 2 : sdl_lib/Couplings & Drives/Flexible Shaft  modelTorsion=true  modelTransverse=false  n_segments=1  parameterization=sdl.enum.shaftParameterization.MaterialProperties  length=flexDLParams.motorMech.shaftOverHang mm  lengths=[1, .5, .25] m  shaft_stiffness=2e5 N*m/rad  shaft_inertia=0.02 kg*m^2  shaft_stiffnesses=[400000, 200000, 100000] N*m/rad  shaft_inertias=[.025, .02, .015] kg*m^2  eiIN=5e5 Pa*m^4  rhoaIN=19 kg/m  eiINs=[600000, 500000, 400000] Pa*m^4  rhoaINs=[20, 19, 18] kg/m  density=7.8e3 kg/m^3  shear_modulus=7.93e9 Pa  elastic_modulus=200e9 Pa  shaft_construction=sdl.enum.shaftConstruction.solid  diameter_outer=flexDLParams.motorMech.bearing2ID mm  diameter_inner=0.05 m  diameter_outers=[.085, .075, .065] m  diameter_inners=[.055, .05, .045] m  damping_ratio=0.01  mu_visc_BF=[0, 0] N*m*s/rad  mu_visc=[0, 0] N*m*s/rad  initial_deflection=0 rad  initial_velocity=0 rpm  num_supports=sdl.enum.num_supports.two  z_support=[0, flexDLParams.motorMech.bearing1Length] mm  boundaryB1=sdl.enum.shaftSupport.clamp  DrotB1_row=[1000, 1000] N*m*s/rad  DtransB1_row=[20000, -44000, -44000, 350000] N*s/m  DtransB1_w_mat=[20000, -44000, -44000, 350000; 10000, -25000, -25000, 140000; 5000, -10000, -10000, 20000] N*s/m  KrotB1_row=[10000, 10000] N*m/rad  KtransB1_row=[1000000, -200000, -300000, 5000000] N/m  KtransB1_w_mat=[1000000, -600000, -3500000, 8000000; 1000000, -200000, -3000000, 5000000; 1000000, -50000, -2500000, 3000000] N/m  boundaryI1=sdl.enum.shaftSupport.clamp  DrotI1_row=[1000, 1000] N*m*s/rad  DtransI1_row=[20000, -44000, -44000, 350000] N*s/m  DtransI1_w_mat=[20000, -44000, -44000, 350000; 10000, -25000, -25000, 140000; 5000, -10000, -10000, 20000] N*s/m  KrotI1_row=[10000, 10000] N*m/rad  KtransI1_row=[1000000, -200000, -300000, 5000000] N/m  KtransI1_w_mat=[1000000, -600000, -3500000, 8000000; 1000000, -200000, -3000000, 5000000; 1000000, -50000, -2500000, 3000000] N/m  boundaryI2=sdl.enum.shaftSupport.clamp  DrotI2_row=[1000, 1000] N*m*s/rad  DtransI2_row=[20000, -44000, -44000, 350000] N*s/m  DtransI2_w_mat=[20000, -44000, -44000, 350000; 10000, -25000, -25000, 140000; 5000, -10000, -10000, 20000] N*s/m  KrotI2_row=[10000, 10000] N*m/rad  KtransI2_row=[1000000, -200000, -300000, 5000000] N/m  KtransI2_w_mat=[1000000, -600000, -3500000, 8000000; 1000000, -200000, -3000000, 5000000; 1000000, -50000, -2500000, 3000000] N/m  boundaryF1=sdl.enum.shaftSupport.clamp  DrotF1_row=[1000, 1000] N*m*s/rad  DtransF1_row=[20000, -44000, -44000, 350000] N*s/m  DtransF1_w_mat=[20000, -44000, -44000, 350000; 10000, -25000, -25000, 140000; 5000, -10000, -10000, 20000] N*s/m  KrotF1_row=[10000, 10000] N*m/rad  KtransF1_row=[1000000, -200000, -300000, 5000000] N/m  KtransF1_w_mat=[1000000, -600000, -3500000, 8000000; 1000000, -200000, -3000000, 5000000; 1000000, -50000, -2500000, 3000000] N/m  bearing_speed=[200, 500, 1500] rpm  alpha=10 1/s  beta=1e-8 s  noDisk=sdl.enum.shaftDisks.none  zDisk=0.5 m  mDiskIN=2 kg  IdDiskIN=0.025 kg*m^2  IpDiskIN=0.050 kg*m^2  enable_static_unbalance=true  offsetMR=[.01, .01] kg*m  offsetMR_initialAngleIN=[0, pi] rad  offsetMassLocation=[.33, .67] m  enable_external_force=false  externalForce=[1, 2] N  externalForceHarmonic=[.5, 2]  externalLoadAngle=[pi / 2, 3 * pi / 4] rad  zExternalLoad=[.25, .75] m  AnalysisMethod=sdl.enum.bendingAnalysisMethod.LumpedMass  ModeInputMethod=sdl.enum.modeInputMethod.SimscapeDetermined  numModesIn=6  mode_speed_dependency=sdl.enum.mode_speed_dependency.Static  OmegaNom=5000 rpm  wMax=1e8 rpm  dz=0.01 m  userMode_w=[280, 644, 615, 1285] rad/s  userMode_w_mat=[257, 780, 580, 1560; 280, 644, 615, 1285; 294, 513, 636, 1020] rad/s  userMode_z=[0, .1, .2, .3, .4, .5, .6, .7, .8, .9, 1] m  userMode_shapeX=[.1648, .0086, -.2759, .0162; .1671, .0093, -.2231, .0133; .1691, .01, -.1689, .0102; .1707, .0105, -.1135, .007; .1717, .0108, -.057, .0035; .1721, .0109, 0, 0; .1717, .0108, .057, -.0035; .1707, .0105, .1135, -.007; .1691, .01, .1689, -.0102; .1671, .0093, .2231, -.0133; .1648, .0086, .2759, -.0162]  userMode_shapeX_mat=cat(3, [.1842, .0134, -.3072, .0272; .1863, .0152, -.2482, .0226; .1882, .0169, -.1878, .0176; .1897, .0182, -.1261, .0121; .1906, .019, -.0634, .0062; .191, .0193, 0, 0; .1906, .019, .0634, -.0062; .1897, .0182, .1261, -.0121; .1882, .0169, .1878, -.0176; .1863, .0152, .2482, -.0226; .1842, .0134, .3072, -.0272], [.1648, .0086, -.2759, .0162; .1671, .0093, -.2231, .0133; .1691, .01, -.1689, .0102; .1707, .0105, -.1135, .007; .1717, .0108, -.057, .0035; .1721, .0109, 0, 0; .1717, .0108, .057, -.0035; .1707, .0105, .1135, -.007; .1691, .01, .1689, -.0102; .1671, .0093, .2231, -.0133; .1648, .0086, .2759, -.0162], [.1291, .0046, -.2166, .0082; .131, .0048, -.1751, .0067; .1327, .005, -.1327, .0051; .1341, .0052, -.0891, .0035; .135, .0053, -.0448, .0017; .1353, .0053, 0, 0; .135, .0053, .0448, -.0017; .1341, .0052, .0891, -.0035; .1327, .005, .1327, -.0051; .131, .0048, .1751, -.0067; .1291, .0046, .2166, -.0082])  userMode_shapeY=[.1193, -.1784, -.1997, -.3348; .1209, -.1933, -.1615, -.2751; .1224, -.2068, -.1223, -.2119; .1235, -.2176, -.0821, -.1445; .1243, -.2245, -.0413, -.0734; .1246, -.2269, 0, 0; .1243, -.2245, .0413, .0734; .1235, -.2176, .0821, .1445; .1224, -.2068, .1223, .2119; .1209, -.1933, .1615, .2751; .1193, -.1784, .1997, .3348]  userMode_shapeY_mat=cat(3, [.0885, -.1625, -.1475, -.3301; .0895, -.1847, -.1192, -.2745; .0904, -.2048, -.0902, -.2141; .0911, -.2209, -.0606, -.1475; .0916, -.2313, -.0304, -.0754; .0917, -.2349, 0, 0; .0916, -.2313, .0304, .0754; .0911, -.2209, .0606, .1475; .0904, -.2048, .0902, .2141; .0895, -.1847, .1192, .2745; .0885, -.1625, .1475, .3301], [.1193, -.1784, -.1997, -.3348; .1209, -.1933, -.1615, -.2751; .1224, -.2068, -.1223, -.2119; .1235, -.2176, -.0821, -.1445; .1243, -.2245, -.0413, -.0734; .1246, -.2269, 0, 0; .1243, -.2245, .0413, .0734; .1235, -.2176, .0821, .1445; .1224, -.2068, .1223, .2119; .1209, -.1933, .1615, .2751; .1193, -.1784, .1997, .3348], [.1566, -.1901, -.2628, -.3377; .1589, -.1994, -.2125, -.2753; .161, -.2079, -.1609, -.2103; .1627, -.2146, -.1081, -.1424; .1638, -.219, -.0544, -.0719; .1642, -.2205, 0, 0; .1638, -.219, .0544, .0719; .1627, -.2146, .1081, .1424; .161, -.2079, .1609, .2103; .1589, -.1994, .2125, .2753; .1566, -.1901, .2628, .3377])  eta_lumped_nominal=1  etaDer_lumped_nominal=1  eta_modal_nominal=1  etaDer_modal_nominal=1
      settings: InternalSimscapePortConfiguration="{\"Bottom\":[],\"Left\":[{\"id\":\"B\",\"label\":\"B\",\"type\":\"foundation.mechanical.rotational.rotational\"}],\"Right\":[{\"id\":\"F\",\"label\":\"F\",\"type\":\"foundation.mechanical.rotational.rotational\"}],\"Top\":[]}"
  Pinion inertia : fl_lib/Mechanical/Rotational Elements/Inertia  inertia=flexDLParams.motor.j*.2 kg*m^2  num_ports=foundation.enum.numPorts2.one  w_specify=on  w_priority=High  w=0 rpm  w_nominal_specify=off  w_nominal_value=1  w_nominal_unit=rad/s  t_specify=off  t_priority=High  t=0 N*m  t_nominal_specify=off  t_nominal_value=1  t_nominal_unit=N*m
  Rotor Iron : fl_lib/Mechanical/Rotational Elements/Inertia  inertia=flexDLParams.motor.j*0.5 kg*m^2  num_ports=foundation.enum.numPorts2.one  w_specify=on  w_priority=High  w=0 rpm  w_nominal_specify=off  w_nominal_value=1  w_nominal_unit=rad/s  t_specify=off  t_priority=High  t=0 N*m  t_nominal_specify=off  t_nominal_value=1  t_nominal_unit=N*m
  TRQ2RadialLoad2 : Subsystem
  I : PMIOPort  Side=Left
  O : PMIOPort  Port=2  Side=Right
  connections:
  TRQ2RadialLoad2/LConn1 -- Ideal Torque Sensor1/RConn2
  Bearing1/LConn2 -- Bearing/LConn2 -- TRQ2RadialLoad2/RConn1
  Bearing/LConn1 -- Motor Shaft 1/LConn1
  Mechanical Rotational Reference2/LConn1 -- Bearing1/RConn2
  Ideal Torque Sensor1/RConn1 -- Bearing1/RConn1
  Motor Shaft 2/LConn1 -- Bearing1/LConn1
  Mechanical Rotational Reference1/LConn1 -- Bearing/RConn1
  O/RConn1 -- Pinion inertia/LConn1 -- Motor Shaft 2/RConn1
  I/RConn1 -- Ideal Torque Sensor1/LConn1 -- Rotor Iron/LConn1 -- Motor Shaft 1/RConn1

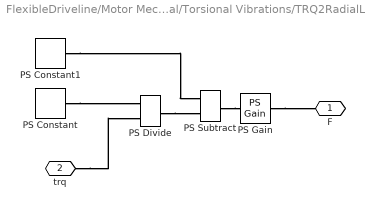
== system FlexibleDriveline/Motor Mechanical/Torsional Vibrations/TRQ2RadialLoad2 ==
  PS Constant : fl_lib/Physical Signals/Sources/PS Constant  constant=25e-3 m
  PS Constant1 : fl_lib/Physical Signals/Sources/PS Constant  constant=5*9.81 N
  PS Divide : fl_lib/Physical Signals/Functions/PS Divide
  PS Gain : fl_lib/Physical Signals/Functions/PS Gain  gain=0.5
  PS Subtract : fl_lib/Physical Signals/Functions/PS Subtract
  F : PMIOPort  Side=Right
  trq : PMIOPort  Port=2  Side=Left
  connections:
  trq/RConn1 -- PS Divide/LConn1
  PS Constant1/RConn1 -- PS Subtract/LConn2
  PS Divide/RConn1 -- PS Subtract/LConn1
  PS Gain/RConn1 -- F/RConn1
  PS Subtract/RConn1 -- PS Gain/LConn1
  PS Constant/RConn1 -- PS Divide/LConn2
